simulink model "Shaddad_GNC"  (R2026b)
undefined symbols (not defined in the file): P, Ts
settings Model: Creator=aomar  LastModifiedBy=aomar

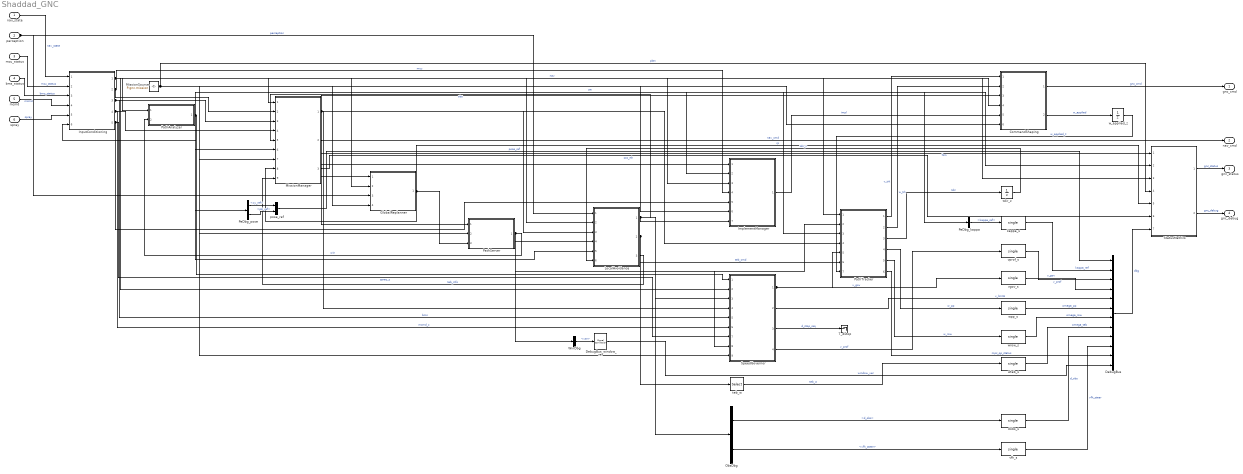
== system Shaddad_GNC ==
  nav_state : Inport  OutDataTypeStr=Bus: Bus_NavState  SampleTime=Ts.ctrl  BusOutputAsStruct=on
  perception : Inport  Port=2  OutDataTypeStr=Bus: Bus_Perception  SampleTime=Ts.hk  BusOutputAsStruct=on
  mcu_status : Inport  Port=3  OutDataTypeStr=Bus: Bus_McuStatus  SampleTime=Ts.comm  BusOutputAsStruct=on
  bms_status : Inport  Port=4  OutDataTypeStr=Bus: Bus_BmsStatus  SampleTime=Ts.hk  BusOutputAsStruct=on
  mcmd : Inport  Port=5  OutDataTypeStr=Bus: Bus_MissionCmd  SampleTime=Ts.gnc_status  BusOutputAsStruct=on
  spray : Inport  Port=6  OutDataTypeStr=Bus: Bus_SprayDemand  SampleTime=Ts.hk  BusOutputAsStruct=on
  CommandShaping : Subsystem  ReferencedSubsystem=gnc_CommandShaping
  DebugBus : BusCreator  Inputs=12  OutDataTypeStr=Bus: Bus_GncDebug  NonVirtualBus=on
  DebugBus_window_ver : SignalConversion  OverrideOpt=off
  GlobalReplanner : Subsystem  ReferencedSubsystem=gnc_GlobalReplanner
  ImplementManager : Subsystem  ReferencedSubsystem=gnc_ImplementManager
  InputConditioning : Subsystem  ReferencedSubsystem=gnc_InputConditioning
  LocalAvoidance : Subsystem  ReferencedSubsystem=gnc_LocalAvoidance
  MissionManager : Subsystem  ReferencedSubsystem=gnc_MissionManager
  MissionSource : Constant  Value=P.gnc.mission  OutDataTypeStr=Bus: Bus_MissionPlan
  ObsDbg : BusSelector  OutputSignals=d_obs,vfh_steer
  PathAnalyzer : Subsystem  ReferencedSubsystem=gnc_PathAnalyzer
  PathServer : Subsystem  ReferencedSubsystem=gnc_PathServer
  PathTracker : Subsystem  ReferencedSubsystem=gnc_PathTracker
  PeDbg_kappa : BusSelector  OutputSignals=kappa_ref
  PeDbg_pose : BusSelector  OutputSignals=xy_ref,psi_ref
  SpeedGovernor : Subsystem  ReferencedSubsystem=gnc_SpeedGovernor
  StatusMetrics : Subsystem  ReferencedSubsystem=gnc_StatusMetrics
  T_dstop : Terminator
  WinDbg : BusSelector  OutputSignals=ver
  dobs_s : DataTypeConversion  OutDataTypeStr=single  RndMeth=Nearest
  kappa_s : DataTypeConversion  OutDataTypeStr=single  RndMeth=Nearest
  pose_ref : Concatenate
  tdir_z : UnitDelay  SampleTime=Ts.gnc
  teb_w : Selector  IndexOptions=Index vector (dialog)  Indices=2  OutputSizes=1
  vfh_s : DataTypeConversion  OutDataTypeStr=single  RndMeth=Nearest
  vgov_s : DataTypeConversion  OutDataTypeStr=single  RndMeth=Nearest
  vprof_s : DataTypeConversion  OutDataTypeStr=single  RndMeth=Nearest
  w_applied_z : UnitDelay  SampleTime=Ts.gnc
  wpp_s : DataTypeConversion  OutDataTypeStr=single  RndMeth=Nearest
  wrow_s : DataTypeConversion  OutDataTypeStr=single  RndMeth=Nearest
  wteb_s : DataTypeConversion  OutDataTypeStr=single  RndMeth=Nearest
  gnc_cmd : Outport  OutDataTypeStr=Bus: Bus_GncCmd  SampleTime=Ts.comm  BusOutputAsStruct=on
  nav_cmd : Outport  Port=2  OutDataTypeStr=Bus: Bus_NavCmd  SampleTime=Ts.comm  BusOutputAsStruct=on
  gnc_status : Outport  Port=3  OutDataTypeStr=Bus: Bus_GncStatus  SampleTime=Ts.gnc_status  BusOutputAsStruct=on
  gnc_debug : Outport  Port=4  OutDataTypeStr=Bus: Bus_GncDebug  SampleTime=Ts.comm  BusOutputAsStruct=on
  wires:
  nav_state/1 -> InputConditioning/1  "nav_state"
  perception/1 -> LocalAvoidance/1, GlobalReplanner/3  "perception"
  mcu_status/1 -> InputConditioning/2  "mcu_status"
  bms_status/1 -> InputConditioning/3  "bms_status"
  mcmd/1 -> InputConditioning/4  "mcmd"
  spray/1 -> InputConditioning/5  "spray"
  InputConditioning/3 -> SpeedGovernor/5, MissionManager/3  "bms"
  MissionSource/1 -> SpeedGovernor/9, PathServer/2, ImplementManager/6, GlobalReplanner/4, StatusMetrics/4, MissionManager/7, CommandShaping/6  "plan"
  PathAnalyzer/1 -> SpeedGovernor/1, LocalAvoidance/5, PathTracker/3, PeDbg_kappa/1, PeDbg_pose/1, ImplementManager/2, StatusMetrics/2, MissionManager/6, InputConditioning/6  "pe"
  PeDbg_pose/1 -> pose_ref/1  "<xy_ref>"
  PeDbg_pose/2 -> pose_ref/2  "<psi_ref>"
  pose_ref/1 -> DebugBus/1  "pose_ref"
  MissionManager/1 -> SpeedGovernor/4, PathTracker/4, LocalAvoidance/3, PathServer/1, GlobalReplanner/1, ImplementManager/1, StatusMetrics/1, CommandShaping/3  "fsm"
  MissionManager/2 -> nav_cmd/1  "nav_cmd"
  MissionManager/3 -> StatusMetrics/6  "soc_rth"
  GlobalReplanner/1 -> PathServer/3, MissionManager/8, StatusMetrics/5  "rp"
  PathServer/1 -> PathAnalyzer/2, SpeedGovernor/8, WinDbg/1, PathTracker/2, LocalAvoidance/4  "win"
  WinDbg/1 -> DebugBus_window_ver/1  "<ver>"
  DebugBus_window_ver/1 -> DebugBus/12  "window_ver"
  LocalAvoidance/3 -> MissionManager/9  "teb_info"
  ObsDbg/1 -> dobs_s/1  "<d_obs>"
  ObsDbg/2 -> vfh_s/1  "<vfh_steer>"
  teb_w/1 -> wteb_s/1  "teb_w"
  ImplementManager/1 -> CommandShaping/5  "impl"
  SpeedGovernor/1 -> PathTracker/5, vgov_s/1  "v_gov"
  SpeedGovernor/2 -> DebugBus/5  "v_limits"
  SpeedGovernor/3 -> T_dstop/1  "d_stop_req"
  SpeedGovernor/4 -> vprof_s/1  "v_prof"
  PathTracker/1 -> CommandShaping/1  "v_trk"
  PathTracker/2 -> CommandShaping/2  "w_trk"
  PathTracker/3 -> tdir_z/1  "tdir"
  PathTracker/4 -> wpp_s/1  "w_pp"
  PathTracker/5 -> wrow_s/1  "w_row"
  PathTracker/6 -> DebugBus/11  "mpc_qp_status"
  PeDbg_kappa/1 -> kappa_s/1  "<kappa_ref>"
  tdir_z/1 -> LocalAvoidance/6  "tdir_z"
  kappa_s/1 -> DebugBus/2  "kappa_ref"
  vprof_s/1 -> DebugBus/3  "v_prof"
  vgov_s/1 -> DebugBus/4  "v_gov"
  wpp_s/1 -> DebugBus/6  "omega_pp"
  wrow_s/1 -> DebugBus/7  "omega_row"
  wteb_s/1 -> DebugBus/8  "omega_teb"
  dobs_s/1 -> DebugBus/9  "d_obs"
  vfh_s/1 -> DebugBus/10  "vfh_steer"
  CommandShaping/1 -> gnc_cmd/1  "gnc_cmd"
  CommandShaping/2 -> w_applied_z/1  "w_applied"
  DebugBus/1 -> StatusMetrics/7  "dbg"
  w_applied_z/1 -> PathTracker/7  "w_applied_z"
  StatusMetrics/1 -> gnc_status/1  "gnc_status"
  StatusMetrics/2 -> gnc_debug/1  "gnc_debug"
  LocalAvoidance/1 -> ObsDbg/1, SpeedGovernor/3, MissionManager/5, ImplementManager/7  "obs"
  LocalAvoidance/2 -> teb_w/1, PathTracker/6  "teb_cmd"
  InputConditioning/4 -> SpeedGovernor/6, MissionManager/4  "mcmd_c"
  InputConditioning/5 -> SpeedGovernor/7, ImplementManager/5  "spray_c"
  InputConditioning/1 -> SpeedGovernor/2, LocalAvoidance/2, PathTracker/1, GlobalReplanner/2, ImplementManager/3, StatusMetrics/3, PathAnalyzer/1, CommandShaping/4, MissionManager/1  "nav"
  InputConditioning/2 -> ImplementManager/4, MissionManager/2  "mcu"
